simulink model "HW6"  (R2022b)
settings: Solver=VariableStepAuto  StartTime=0.0  StopTime=10  FixedStep=0.01  RelTol=1e-3
libraries: simulink x1
settings Model: Creator=ali14  LastModifiedBy=ali14

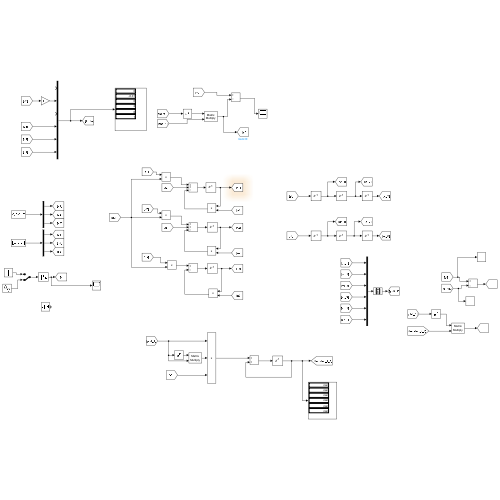
[thumbnail: Simulink's stored preview of the top-level diagram]
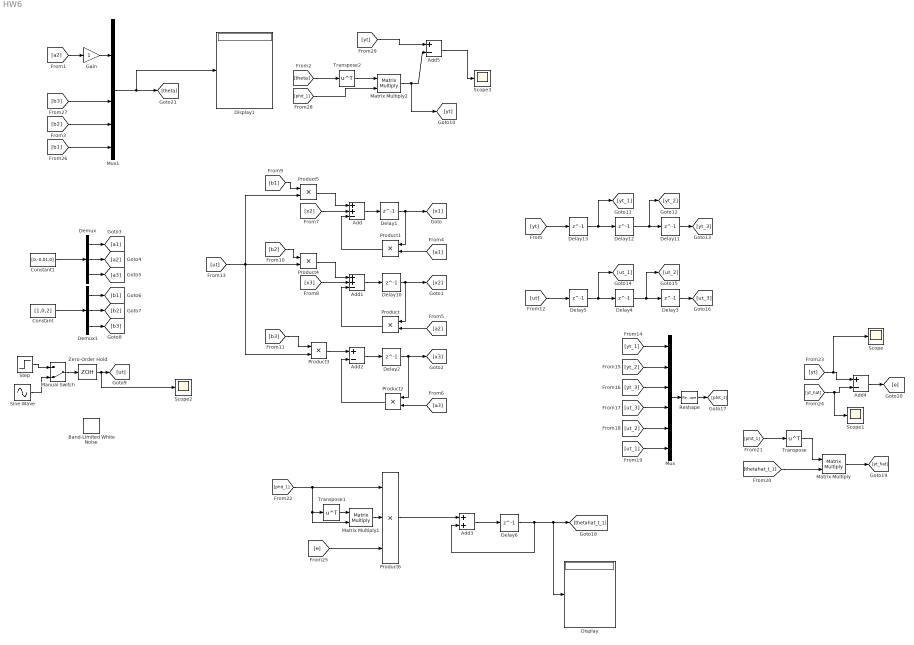
== system HW6 ==
  Add : Sum  Inputs=++-
  Add1 : Sum  Inputs=++-
  Add2 : Sum  Inputs=+-
  Add3 : Sum
  Add4 : Sum  Inputs=+-
  Add5 : Sum  Inputs=+-
  Band-Limited White Noise : simulink/Sources/Band-Limited White Noise  Cov=[0.1]  Ts=0.01  seed=[23341]
  Constant : Constant  Value=[1,0,2]
  Constant1 : Constant  Value=[0,-0.01,0]
  Delay{1..5,10..13} (9 alike) : Delay  DelayLength=1  SampleTime=0.01
  Delay6 : Delay  DelayLength=1  InitialCondition=0  SampleTime=0.01
  Demux : Demux  Outputs=3
  Demux1 : Demux  Outputs=3
  Display : Display
  Display1 : Display
      settings: Decimation=2
  Gain : Gain
  Manual Switch : ManualSwitch  CurrentSetting=0
  Matrix Multiply : Product  Multiplication=Matrix(*)
  Matrix Multiply1 : Product  Multiplication=Matrix(*)
  Matrix Multiply2 : Product  Multiplication=Matrix(*)
  Mux : Mux  Inputs=6
  Mux1 : Mux  Inputs=6
  Product{,1..5} (6 alike) : Product
  Product6 : Product  Inputs=3
  Reshape : Reshape  OutputDimensionality=Column vector (2-D)
  Scope{,1..3} (4 alike) : Scope
  Sine Wave : Sin  SampleTime=0
  Step : Step  SampleTime=0
  Transpose : Math  Operator=transpose
  Transpose1 : Math  Operator=transpose
  Transpose2 : Math  Operator=transpose
  Zero-Order Hold : ZeroOrderHold  SampleTime=0.01
  wires:
  Add1/1 -> Delay10/1
  Delay1/1 -> Product1/1, [x1]
  Delay10/1 -> Product/1, [x2]
  Product1/1 -> Add/3
  Product/1 -> Add1/3
  Add2/1 -> Delay2/1
  Delay2/1 -> Product2/1, [x3]
  Product2/1 -> Add2/2
  [a1] -> Product1/2
  [a2] -> Product/2
  [a3] -> Product2/2
  [x2] -> Add/2
  [x3] -> Add1/2
  Product3/1 -> Add2/1
  Product4/1 -> Add1/1
  Product5/1 -> Add/1
  [b1] -> Product5/1
  [b3] -> Product3/1
  [b2] -> Product4/1
  Constant1/1 -> Demux/1
  Constant/1 -> Demux1/1
  Demux/1 -> [a1]
  Demux/2 -> [a2]
  Demux/3 -> [a3]
  Demux1/1 -> [b1]
  Demux1/2 -> [b2]
  Demux1/3 -> [b3]
  [ut] -> Product3/2, Product4/2, Product5/2
  [yt] -> Delay13/1
  Delay13/1 -> Delay12/1, [yt_1]
  Delay12/1 -> Delay11/1, [yt_2]
  Delay11/1 -> [yt_3]
  Zero-Order Hold/1 -> Scope2/1, [ut]
  Delay4/1 -> Delay3/1, [ut_2]
  Delay5/1 -> Delay4/1, [ut_1]
  [ut] -> Delay5/1
  Delay3/1 -> [ut_3]
  Mux/1 -> Reshape/1
  [yt_1] -> Mux/1
  [yt_2] -> Mux/2
  [yt_3] -> Mux/3
  [ut_3] -> Mux/4
  [ut_2] -> Mux/5
  [ut_1] -> Mux/6
  Reshape/1 -> [phit_1]
  Add3/1 -> Delay6/1
  Delay6/1 -> [thetahat_t_1], Display/1, Add3/2
  [phit_1] -> Transpose/1
  Transpose/1 -> Matrix Multiply/1
  [thetahat_t_1] -> Matrix Multiply/2
  Matrix Multiply/1 -> [yt_hat]
  [phit_1] -> Matrix Multiply1/2, Transpose1/1, Product6/1
  Transpose1/1 -> Matrix Multiply1/1
  [yt] -> Scope/1, Add4/1
  Add4/1 -> [e]
  [yt_hat] -> Scope1/1, Add4/2
  [e] -> Product6/3
  Matrix Multiply1/1 -> Product6/2
  Manual Switch/1 -> Zero-Order Hold/1
  Step/1 -> Manual Switch/1
  Sine Wave/1 -> Manual Switch/2
  Product6/1 -> Add3/1
  Add/1 -> Delay1/1
  Mux1/1 -> Display1/1, [theta]
  Gain/1 -> Mux1/2
  [b1] -> Mux1/6
  [b2] -> Mux1/5
  [b3] -> Mux1/4
  [a2] -> Gain/1
  [theta] -> Transpose2/1
  Transpose2/1 -> Matrix Multiply2/1
  Matrix Multiply2/1 -> [yt], Add5/2
  [phit_1] -> Matrix Multiply2/2
  [yt] -> Add5/1
  Add5/1 -> Scope3/1
